simulink model "interfacage_spi"  (Simulink 7.0)
settings: Solver=FixedStepDiscrete  StartTime=0.0  StopTime=10.0  FixedStep=0.01  RelTol=1e-3
libraries: dsPICdrivers x8, simulink x2
settings Model: Creator=Administrator  LastModifiedBy=Administrator
settings OptimizationCC: OptimizeModelRefInitCode=on  LifeSpan=1
settings HardwareCC: ProdBitPerInt=16  ProdEndianess=LittleEndian  ProdWordSize=16  ProdHWDeviceType=16-bit Generic
settings RTWCC: SystemTargetFile=dspic.tlc  TemplateMakefile=dspic_pic30_gcc.tmf  PostCodeGenCommand=dsPIC_Compile()  Description=Embedded Target for Microchip dsPIC (real-time)  ProcessScript=dspic_make_rtw_hook
settings CodeAppCC: IgnoreCustomStorageClasses=off
settings STFCustomTargetCC: GenFloatMathFcnCalls=ANSI_C  ModelReferenceCompliant=off  IncludeMdlTerminateFcn=off  CombineOutputUpdateFcns=on  SuppressErrorStatus=on  ERTCustomFileBanners=on  SupportContinuousTime=off  SupportNonInlinedSFcns=off  SystemTargetFile=dspic.tlc
settings ERTTargetCC: GenFloatMathFcnCalls=ANSI_C  ModelReferenceCompliant=off  CompOptLevelCompliant=off  IncludeMdlTerminateFcn=off  SuppressErrorStatus=on  ModelStepFunctionPrototypeControlCompliant=off  ExtModeMexFile=noextcomm  InlinedParameterPlacement=NonHierarchical  ERTSrcFileBannerTemplate=dsPIC_code_template.cgt  ERTHdrFileBannerTemplate=dsPIC_code_template.cgt  ERTDataSrcFileTemplate=dsPIC_code_template.cgt  ERTDataHdrFileTemplate=dsPIC_code_template.cgt  ERTCustomFileTemplate=dsPIC_main.tlc
settings CustomProperty: DataType=string  Value=C:\PROGRA~1\MATLAB\R2007b\bin\win32\gmake

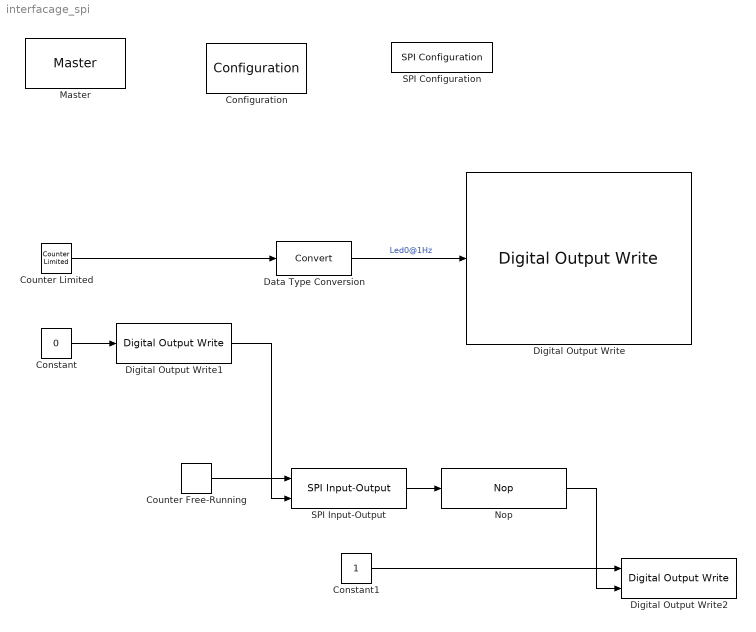
== system interfacage_spi ==
  Configuration : dsPICdrivers/Configuration  SystemSampleTime=-1  double64=on
  Constant : Constant  Value=0  OutDataTypeMode=boolean  OutDataType=sfix(16)  OutScaling=2^0
  Constant1 : Constant  OutDataTypeMode=boolean  OutDataType=sfix(16)  OutScaling=2^0
  Counter Free-Running : simulink/Sources/Counter Free-Running  SystemSampleTime=-1  NumBits=16  tsamp=-1
  Counter Limited : simulink/Sources/Counter Limited  SystemSampleTime=-1  uplimit=1  tsamp=-1
  Data Type Conversion : DataTypeConversion  OutDataTypeMode=boolean  OutDataType=sfix(16)  OutScaling=2^0
  Digital Output Write : dsPICdrivers/Digital I//O/Digital Output Write  Tag=dsPIC_Digital_Output  Priority=5  PORT=A  Pin=[0]  Simultaneous=off  OrderingInOutPopup=None
  Digital Output Write1 : dsPICdrivers/Digital I//O/Digital Output Write  Tag=dsPIC_Digital_Output  Priority=5  PORT=A  Pin=[1]  Simultaneous=off  OrderingInOutPopup=Output
  Digital Output Write2 : dsPICdrivers/Digital I//O/Digital Output Write  Tag=dsPIC_Digital_Output  Priority=5  PORT=A  Pin=[1]  Simultaneous=off  OrderingInOutPopup=Input
  Master : dsPICdrivers/Master  Tag=dsPIC_MASTER  Priority=1  TimeStepType=Timer1  picType=33fJ256GP710  fcy=4000000  Quartz_33f=8e6  PLLActive_33f=off  fcyDesired_33f=0  tmr1="[1  39999  0]"  tmr1Info="Time Step : 0.01  ;   Error : 0%  PR1=39999"  tmr2345="[0  0  0  0  0  0  0  0]"  tmr2345cfg=[-1 -1 -1 -1 -1 -1 -1 -1]  IOautoConf=on  typePort="[ 10  10   0   0   0   0   0   0   0   0   0   0   0   0   0   0   0   0   0   0   0   0   0   0   0   0   0   0   0   0   0   0   0   0   0   0   0   0   0   0   0   0   0   0   0   0   0   0   0   0   0   0   0   0   0   0   0   0   0   0   0   0   0   0   0   0   0   0   0   0   0   0   0   0   0   0   0   0   0   0   0   0   0   0   0   0  17  14  15   0   0   0   0   0   0   0   0   0   0   0   0   0   0   0   0   0   0   0   0   0   0   0 ]"  TRIS="[ 65532  65535  65535  65535  65535  65535  65535 ]"  ADPCFG=0  MasterBusyPort=None  MasterOverloadPort=None  FOSC=Quartz (XT - HS)  TempProtection_33f=TEMP_ON  FPBOR=<empty>  PWRT=disable  MCLR=<empty>  PowerSave=off
  Nop : dsPICdrivers/OTHERS/Nop  Tag=dsPIC_Reset  NbrNop=500
  SPI Configuration : dsPICdrivers/SPI PORT/SPI Configuration  Tag=dsPIC_config_SPI  Priority=2  ConfigurationTime=At boot time (only once)  OrderingInOutPopup=None  SampleTime=-1  Frame_Enable=0  Frame_Sync=None  SPI=1  MODE=MASTER  USER_SCALER=12  StartEnable=Enable  SDO_EN=on  DATA_LENGTH=16 bits  SS_EN=off  SMP=End of bit  CKP=high  CKE=Active to Idle  Status="OK - Mode 0  -    Fsck= 333333.3333Hz"
  SPI Input-Output : dsPICdrivers/SPI PORT/SPI Input-Output  Tag=dsPIC_SPI  SPI=1  INPUT=off  RESET_INPUT=on  OUTPUT=on  SPECIAL_SPI=Always Enable  DATA_LENGTH=16 bits  WAIT_INPUTDATA=off  OrderingInOutPopup=Input & Output  SampleTime=-1
  wires:
  Counter Limited/1 -> Data Type Conversion/1
  Data Type Conversion/1 -> Digital Output Write/1  "Led0@1Hz"
  Counter Free-Running/1 -> SPI Input-Output/1
  Digital Output Write1/1 -> SPI Input-Output/2
  Constant/1 -> Digital Output Write1/1
  Constant1/1 -> Digital Output Write2/1
  SPI Input-Output/1 -> Nop/1
  Nop/1 -> Digital Output Write2/2
